simulink model "s_c_nbe_m1k"  (R2016b)
settings: Solver=VariableStepAuto  StartTime=0.0  StopTime=1000  RelTol=1e-3  EnableMultiTasking=on
undefined symbols (not defined in the file): Coeffs, fft_stages, n_taps, output_bits, pfb_coeff_gen_calc, xengbits
libraries: xbsIndex_r4 x23639, casper_library_misc x65, casper_library_scopes x4, xbsReplacements_r4 x4, xps_library x3
(part 142 of 198)

== system s_c_nbe_m1k/DDC/dec_fir_async2/fir_col_async8/fir_tap7 ==
  a : Inport
  b : Inport  Port=2
  c : Inport  Port=3
  d : Inport  Port=4
  dv_in : Inport  Port=5
  AddSub0 : xbsIndex_r4/AddSub  mode=Addition  use_carryin=off  use_carryout=off  en=off  latency=add_latency  precision=Full  arith_type="Signed  (2's comp)"  n_bits=18  bin_pt=16  quantization=Truncate  overflow=Wrap  use_behavioral_HDL=on  hw_selection=Fabric  pipelined=off  use_rpm=on  dbl_ovrd=off  block_type=addsub
  AddSub1 : xbsIndex_r4/AddSub  mode=Addition  use_carryin=off  use_carryout=off  en=off  latency=add_latency  precision=Full  arith_type="Signed  (2's comp)"  n_bits=18  bin_pt=16  quantization=Truncate  overflow=Wrap  use_behavioral_HDL=on  hw_selection=Fabric  pipelined=off  use_rpm=on  dbl_ovrd=off  block_type=addsub
  Mult0 : xbsIndex_r4/Mult  precision=Full  arith_type="Signed  (2's comp)"  n_bits=18  bin_pt=17  quantization=Truncate  overflow=Wrap  en=off  latency=mult_latency  use_behavioral_HDL=on  opt=Speed  use_embedded=on  optimum_pipeline=off  pipeline=on  dbl_ovrd=off  use_rpm=off  placement_style=Rectangular shape  block_type=mult
  Mult1 : xbsIndex_r4/Mult  precision=Full  arith_type="Signed  (2's comp)"  n_bits=18  bin_pt=17  quantization=Truncate  overflow=Wrap  en=off  latency=mult_latency  use_behavioral_HDL=on  opt=Speed  use_embedded=on  optimum_pipeline=off  pipeline=on  dbl_ovrd=off  use_rpm=off  placement_style=Rectangular shape  block_type=mult
  Register{0..3} (4 alike) : xbsIndex_r4/Register  init=0  rst=off  en=on  dbl_ovrd=off  block_type=register
  coefficient : xbsIndex_r4/Constant  const=factor  gui_display_data_type=Fixed-point  arith_type=Signed (2's comp)  n_bits=coeff_bit_width  bin_pt=coeff_bin_pt  preci_type=Single  exp_width=8  frac_width=24  explicit_period=on  period=1  equ=P=C  opselect=C  inp2=PCIN>>17  opr=+  inp1=P  carry=CIN  dbl_ovrd=off  block_type=constant
  a_out : Outport
  b_out : Outport  Port=2
  c_out : Outport  Port=3
  d_out : Outport  Port=4
  real : Outport  Port=5
  imag : Outport  Port=6
  wires:
  dv_in/1 -> Register0/2, Register1/2, Register2/2, Register3/2
  d/1 -> AddSub1/2, Register3/1
  c/1 -> AddSub0/2, Register2/1
  b/1 -> AddSub1/1, Register1/1
  a/1 -> AddSub0/1, Register0/1
  Register0/1 -> a_out/1
  Register1/1 -> b_out/1
  Register2/1 -> c_out/1
  coefficient/1 -> Mult0/1, Mult1/1
  Register3/1 -> d_out/1
  AddSub0/1 -> Mult0/2
  Mult0/1 -> real/1
  AddSub1/1 -> Mult1/2
  Mult1/1 -> imag/1

== system s_c_nbe_m1k/DDC/dec_fir_async2/fir_col_async8/fir_tap8 ==
  a : Inport
  b : Inport  Port=2
  c : Inport  Port=3
  d : Inport  Port=4
  dv_in : Inport  Port=5
  AddSub0 : xbsIndex_r4/AddSub  mode=Addition  use_carryin=off  use_carryout=off  en=off  latency=add_latency  precision=Full  arith_type="Signed  (2's comp)"  n_bits=18  bin_pt=16  quantization=Truncate  overflow=Wrap  use_behavioral_HDL=on  hw_selection=Fabric  pipelined=off  use_rpm=on  dbl_ovrd=off  block_type=addsub
  AddSub1 : xbsIndex_r4/AddSub  mode=Addition  use_carryin=off  use_carryout=off  en=off  latency=add_latency  precision=Full  arith_type="Signed  (2's comp)"  n_bits=18  bin_pt=16  quantization=Truncate  overflow=Wrap  use_behavioral_HDL=on  hw_selection=Fabric  pipelined=off  use_rpm=on  dbl_ovrd=off  block_type=addsub
  Mult0 : xbsIndex_r4/Mult  precision=Full  arith_type="Signed  (2's comp)"  n_bits=18  bin_pt=17  quantization=Truncate  overflow=Wrap  en=off  latency=mult_latency  use_behavioral_HDL=on  opt=Speed  use_embedded=on  optimum_pipeline=off  pipeline=on  dbl_ovrd=off  use_rpm=off  placement_style=Rectangular shape  block_type=mult
  Mult1 : xbsIndex_r4/Mult  precision=Full  arith_type="Signed  (2's comp)"  n_bits=18  bin_pt=17  quantization=Truncate  overflow=Wrap  en=off  latency=mult_latency  use_behavioral_HDL=on  opt=Speed  use_embedded=on  optimum_pipeline=off  pipeline=on  dbl_ovrd=off  use_rpm=off  placement_style=Rectangular shape  block_type=mult
  Register{0..3} (4 alike) : xbsIndex_r4/Register  init=0  rst=off  en=on  dbl_ovrd=off  block_type=register
  coefficient : xbsIndex_r4/Constant  const=factor  gui_display_data_type=Fixed-point  arith_type=Signed (2's comp)  n_bits=coeff_bit_width  bin_pt=coeff_bin_pt  preci_type=Single  exp_width=8  frac_width=24  explicit_period=on  period=1  equ=P=C  opselect=C  inp2=PCIN>>17  opr=+  inp1=P  carry=CIN  dbl_ovrd=off  block_type=constant
  a_out : Outport
  b_out : Outport  Port=2
  c_out : Outport  Port=3
  d_out : Outport  Port=4
  real : Outport  Port=5
  imag : Outport  Port=6
  wires:
  dv_in/1 -> Register0/2, Register1/2, Register2/2, Register3/2
  d/1 -> AddSub1/2, Register3/1
  c/1 -> AddSub0/2, Register2/1
  b/1 -> AddSub1/1, Register1/1
  a/1 -> AddSub0/1, Register0/1
  Register0/1 -> a_out/1
  Register1/1 -> b_out/1
  Register2/1 -> c_out/1
  coefficient/1 -> Mult0/1, Mult1/1
  Register3/1 -> d_out/1
  AddSub0/1 -> Mult0/2
  Mult0/1 -> real/1
  AddSub1/1 -> Mult1/2
  Mult1/1 -> imag/1

== system s_c_nbe_m1k/DDC/dec_fir_async2/fir_col_async8/fir_tap9 ==
  a : Inport
  b : Inport  Port=2
  c : Inport  Port=3
  d : Inport  Port=4
  dv_in : Inport  Port=5
  AddSub0 : xbsIndex_r4/AddSub  mode=Addition  use_carryin=off  use_carryout=off  en=off  latency=add_latency  precision=Full  arith_type="Signed  (2's comp)"  n_bits=18  bin_pt=16  quantization=Truncate  overflow=Wrap  use_behavioral_HDL=on  hw_selection=Fabric  pipelined=off  use_rpm=on  dbl_ovrd=off  block_type=addsub
  AddSub1 : xbsIndex_r4/AddSub  mode=Addition  use_carryin=off  use_carryout=off  en=off  latency=add_latency  precision=Full  arith_type="Signed  (2's comp)"  n_bits=18  bin_pt=16  quantization=Truncate  overflow=Wrap  use_behavioral_HDL=on  hw_selection=Fabric  pipelined=off  use_rpm=on  dbl_ovrd=off  block_type=addsub
  Mult0 : xbsIndex_r4/Mult  precision=Full  arith_type="Signed  (2's comp)"  n_bits=18  bin_pt=17  quantization=Truncate  overflow=Wrap  en=off  latency=mult_latency  use_behavioral_HDL=on  opt=Speed  use_embedded=on  optimum_pipeline=off  pipeline=on  dbl_ovrd=off  use_rpm=off  placement_style=Rectangular shape  block_type=mult
  Mult1 : xbsIndex_r4/Mult  precision=Full  arith_type="Signed  (2's comp)"  n_bits=18  bin_pt=17  quantization=Truncate  overflow=Wrap  en=off  latency=mult_latency  use_behavioral_HDL=on  opt=Speed  use_embedded=on  optimum_pipeline=off  pipeline=on  dbl_ovrd=off  use_rpm=off  placement_style=Rectangular shape  block_type=mult
  Register{0..3} (4 alike) : xbsIndex_r4/Register  init=0  rst=off  en=on  dbl_ovrd=off  block_type=register
  coefficient : xbsIndex_r4/Constant  const=factor  gui_display_data_type=Fixed-point  arith_type=Signed (2's comp)  n_bits=coeff_bit_width  bin_pt=coeff_bin_pt  preci_type=Single  exp_width=8  frac_width=24  explicit_period=on  period=1  equ=P=C  opselect=C  inp2=PCIN>>17  opr=+  inp1=P  carry=CIN  dbl_ovrd=off  block_type=constant
  a_out : Outport
  b_out : Outport  Port=2
  c_out : Outport  Port=3
  d_out : Outport  Port=4
  real : Outport  Port=5
  imag : Outport  Port=6
  wires:
  dv_in/1 -> Register0/2, Register1/2, Register2/2, Register3/2
  d/1 -> AddSub1/2, Register3/1
  c/1 -> AddSub0/2, Register2/1
  b/1 -> AddSub1/1, Register1/1
  a/1 -> AddSub0/1, Register0/1
  Register0/1 -> a_out/1
  Register1/1 -> b_out/1
  Register2/1 -> c_out/1
  coefficient/1 -> Mult0/1, Mult1/1
  Register3/1 -> d_out/1
  AddSub0/1 -> Mult0/2
  Mult0/1 -> real/1
  AddSub1/1 -> Mult1/2
  Mult1/1 -> imag/1

== system s_c_nbe_m1k/DDC/dec_fir_async3/convert_of/convert ==
  note: (ones_bit & 1) -> round-to-even
      | (ones_bit ^ 1) -> round-to-odd
      | (sign_bit & 1)-> round-to-zero
      | (sign_bit ^ 1) -> round-to-inf
      | (X ~| 1) -> round half down
      | (X | 1) -> round half up
  in : Inport
  Concat : xbsIndex_r4/Concat  num_inputs=2  dbl_ovrd=off  block_type=concat
      settings: block_version=10.1.3
  Constant : xbsIndex_r4/Constant  const=1  gui_display_data_type=Fixed-point  arith_type=Unsigned  n_bits=1  bin_pt=0  preci_type=Single  exp_width=8  frac_width=24  explicit_period=off  period=1  equ=P=C  opselect=C  inp2=PCIN>>17  opr=+  inp1=P  carry=CIN  dbl_ovrd=off  block_type=constant
  Reinterpret : xbsIndex_r4/Reinterpret  force_arith_type=on  arith_type=Unsigned  force_bin_pt=on  bin_pt=0  block_type=reinterpret
      settings: infoedit="Changes signal type without altering the binary representation.   You can changed the signal between signed and unsigned, and relocate the binary point.<P><P>Hardware notes: In hardware this block costs nothing.<P><P>Example:  Suppose the input is 6 bits wide, signed, with 2 fractional bits, and the output is forced to unsigned with 0 fractional bits.  Then an input of -2.0 (1110.00 in binary 2's complement) becomes an output of 56 (111000 in binary)."  block_version=10.1.3
  adder : xbsIndex_r4/AddSub  mode=Addition  use_carryin=off  use_carryout=off  en=off  latency=2  precision=User Defined  arith_type="Signed  (2's comp)"  n_bits=18  bin_pt=17  quantization=Truncate  overflow=Saturate  use_behavioral_HDL=off  hw_selection=Fabric  pipelined=on  use_rpm=on  dbl_ovrd=off  block_type=addsub
      settings: xl_area=[0, 0, 0, 0, 0, 0, 0]  block_version=10.1.3
  almost_half : xbsIndex_r4/Constant  const=131071  gui_display_data_type=Fixed-point  arith_type=Unsigned  n_bits=35  bin_pt=0  preci_type=Single  exp_width=8  frac_width=24  explicit_period=off  period=1  equ=P=C  opselect=C  inp2=PCIN>>17  opr=+  inp1=P  carry=CIN  dbl_ovrd=off  block_type=constant
  bit : xbsIndex_r4/Slice  nbits=1  boolean_output=off  mode=Lower Bit Location + Width  bit1=0  base1=MSB of Input  bit0=0  base0=MSB of Input  dbl_ovrd=off  block_type=slice
      settings: infoedit="Extracts a given range of bits from each input sample and presents it at the output.  The output type is ordinarily unsigned with binary point at zero, but can be Boolean when the slice is one bit wide.<P><P>Hardware notes: In hardware this block costs nothing."  block_version=10.1.3
  force1 : xbsIndex_r4/Reinterpret  force_arith_type=on  arith_type="Signed  (2's comp)"  force_bin_pt=on  bin_pt=35  block_type=reinterpret
      settings: infoedit="Changes signal type without altering the binary representation.   You can changed the signal between signed and unsigned, and relocate the binary point.<P><P>Hardware notes: In hardware this block costs nothing.<P><P>Example:  Suppose the input is 6 bits wide, signed, with 2 fractional bits, and the output is forced to unsigned with 0 fractional bits.  Then an input of -2.0 (1110.00 in binary 2's complement) becomes an output of 56 (111000 in binary)."  block_version=10.1.3
  force2 : xbsIndex_r4/Reinterpret  force_arith_type=off  arith_type="Signed  (2's comp)"  force_bin_pt=on  bin_pt=35  block_type=reinterpret
      settings: infoedit="Changes signal type without altering the binary representation.   You can changed the signal between signed and unsigned, and relocate the binary point.<P><P>Hardware notes: In hardware this block costs nothing.<P><P>Example:  Suppose the input is 6 bits wide, signed, with 2 fractional bits, and the output is forced to unsigned with 0 fractional bits.  Then an input of -2.0 (1110.00 in binary 2's complement) becomes an output of 56 (111000 in binary)."  block_version=10.1.3
  tweak_op : xbsIndex_r4/Logical  logical_function=XOR  inputs=2  en=off  latency=0  precision=Full  arith_type=Unsigned  n_bits=8  bin_pt=2  align_bp=on  dbl_ovrd=off  block_type=logical
      settings: xl_area=[0, 0, 0, 0, 0, 0, 0]
  out : Outport
  wires:
  adder/1 -> out/1
  force2/1 -> adder/2
  force1/1 -> adder/1
  Reinterpret/1 -> Concat/1
  Concat/1 -> force1/1
  in/1 -> bit/1, Reinterpret/1
  almost_half/1 -> force2/1
  bit/1 -> tweak_op/1
  Constant/1 -> tweak_op/2
  tweak_op/1 -> Concat/2

== system s_c_nbe_m1k/DDC/dec_fir_async3/convert_of1/convert ==
  note: (ones_bit & 1) -> round-to-even
      | (ones_bit ^ 1) -> round-to-odd
      | (sign_bit & 1)-> round-to-zero
      | (sign_bit ^ 1) -> round-to-inf
      | (X ~| 1) -> round half down
      | (X | 1) -> round half up
  in : Inport
  Concat : xbsIndex_r4/Concat  num_inputs=2  dbl_ovrd=off  block_type=concat
      settings: block_version=10.1.3
  Constant : xbsIndex_r4/Constant  const=1  gui_display_data_type=Fixed-point  arith_type=Unsigned  n_bits=1  bin_pt=0  preci_type=Single  exp_width=8  frac_width=24  explicit_period=off  period=1  equ=P=C  opselect=C  inp2=PCIN>>17  opr=+  inp1=P  carry=CIN  dbl_ovrd=off  block_type=constant
  Reinterpret : xbsIndex_r4/Reinterpret  force_arith_type=on  arith_type=Unsigned  force_bin_pt=on  bin_pt=0  block_type=reinterpret
      settings: infoedit="Changes signal type without altering the binary representation.   You can changed the signal between signed and unsigned, and relocate the binary point.<P><P>Hardware notes: In hardware this block costs nothing.<P><P>Example:  Suppose the input is 6 bits wide, signed, with 2 fractional bits, and the output is forced to unsigned with 0 fractional bits.  Then an input of -2.0 (1110.00 in binary 2's complement) becomes an output of 56 (111000 in binary)."  block_version=10.1.3
  adder : xbsIndex_r4/AddSub  mode=Addition  use_carryin=off  use_carryout=off  en=off  latency=2  precision=User Defined  arith_type="Signed  (2's comp)"  n_bits=18  bin_pt=17  quantization=Truncate  overflow=Saturate  use_behavioral_HDL=off  hw_selection=Fabric  pipelined=on  use_rpm=on  dbl_ovrd=off  block_type=addsub
      settings: xl_area=[0, 0, 0, 0, 0, 0, 0]  block_version=10.1.3
  almost_half : xbsIndex_r4/Constant  const=131071  gui_display_data_type=Fixed-point  arith_type=Unsigned  n_bits=35  bin_pt=0  preci_type=Single  exp_width=8  frac_width=24  explicit_period=off  period=1  equ=P=C  opselect=C  inp2=PCIN>>17  opr=+  inp1=P  carry=CIN  dbl_ovrd=off  block_type=constant
  bit : xbsIndex_r4/Slice  nbits=1  boolean_output=off  mode=Lower Bit Location + Width  bit1=0  base1=MSB of Input  bit0=0  base0=MSB of Input  dbl_ovrd=off  block_type=slice
      settings: infoedit="Extracts a given range of bits from each input sample and presents it at the output.  The output type is ordinarily unsigned with binary point at zero, but can be Boolean when the slice is one bit wide.<P><P>Hardware notes: In hardware this block costs nothing."  block_version=10.1.3
  force1 : xbsIndex_r4/Reinterpret  force_arith_type=on  arith_type="Signed  (2's comp)"  force_bin_pt=on  bin_pt=35  block_type=reinterpret
      settings: infoedit="Changes signal type without altering the binary representation.   You can changed the signal between signed and unsigned, and relocate the binary point.<P><P>Hardware notes: In hardware this block costs nothing.<P><P>Example:  Suppose the input is 6 bits wide, signed, with 2 fractional bits, and the output is forced to unsigned with 0 fractional bits.  Then an input of -2.0 (1110.00 in binary 2's complement) becomes an output of 56 (111000 in binary)."  block_version=10.1.3
  force2 : xbsIndex_r4/Reinterpret  force_arith_type=off  arith_type="Signed  (2's comp)"  force_bin_pt=on  bin_pt=35  block_type=reinterpret
      settings: infoedit="Changes signal type without altering the binary representation.   You can changed the signal between signed and unsigned, and relocate the binary point.<P><P>Hardware notes: In hardware this block costs nothing.<P><P>Example:  Suppose the input is 6 bits wide, signed, with 2 fractional bits, and the output is forced to unsigned with 0 fractional bits.  Then an input of -2.0 (1110.00 in binary 2's complement) becomes an output of 56 (111000 in binary)."  block_version=10.1.3
  tweak_op : xbsIndex_r4/Logical  logical_function=XOR  inputs=2  en=off  latency=0  precision=Full  arith_type=Unsigned  n_bits=8  bin_pt=2  align_bp=on  dbl_ovrd=off  block_type=logical
      settings: xl_area=[0, 0, 0, 0, 0, 0, 0]
  out : Outport
  wires:
  tweak_op/1 -> Concat/2
  Constant/1 -> tweak_op/2
  bit/1 -> tweak_op/1
  almost_half/1 -> force2/1
  in/1 -> Reinterpret/1, bit/1
  Concat/1 -> force1/1
  Reinterpret/1 -> Concat/1
  force1/1 -> adder/1
  force2/1 -> adder/2
  adder/1 -> out/1

== system s_c_nbe_m1k/DDC/dec_fir_async3/fir_col_async1/adder_tree1 ==
  sync : Inport
  din1 : Inport  Port=2
  din2 : Inport  Port=3
  din3 : Inport  Port=4
  din4 : Inport  Port=5
  din5 : Inport  Port=6
  din6 : Inport  Port=7
  din7 : Inport  Port=8
  din8 : Inport  Port=9
  din9 : Inport  Port=10
  din10 : Inport  Port=11
  din11 : Inport  Port=12
  din12 : Inport  Port=13
  din13 : Inport  Port=14
  din14 : Inport  Port=15
  din15 : Inport  Port=16
  din16 : Inport  Port=17
  addr{1..8} (8 alike) : xbsIndex_r4/AddSub  mode=Addition  use_carryin=off  use_carryout=off  en=off  latency=7  precision=Full  arith_type=Unsigned  n_bits=16  bin_pt=14  quantization=Truncate  overflow=Wrap  use_behavioral_HDL=on  hw_selection=DSP48  pipelined=on  use_rpm=on  dbl_ovrd=off  block_type=addsub
  addr{9..15} (7 alike) : xbsIndex_r4/AddSub  mode=Addition  use_carryin=off  use_carryout=off  en=off  latency=7  precision=Full  arith_type=Unsigned  n_bits=16  bin_pt=14  quantization=Truncate  overflow=Wrap  use_behavioral_HDL=off  hw_selection=DSP48  pipelined=on  use_rpm=on  dbl_ovrd=off  block_type=addsub
  sync_delay : xbsIndex_r4/Delay  rst=off  infoeditControl=Selection of Reset will increase slice count due to use of real FFs and instead of SRLs  en=off  latency=28  reg_retiming=on  dbl_ovrd=off  block_type=delay
      settings: block_version=11.4
  sync_out : Outport
  dout : Outport  Port=2
  wires:
  addr15/1 -> dout/1
  addr14/1 -> addr15/2
  addr13/1 -> addr15/1
  addr12/1 -> addr14/2
  addr11/1 -> addr14/1
  addr10/1 -> addr13/2
  addr9/1 -> addr13/1
  addr8/1 -> addr12/2
  addr7/1 -> addr12/1
  addr6/1 -> addr11/2
  addr5/1 -> addr11/1
  addr4/1 -> addr10/2
  addr3/1 -> addr10/1
  addr2/1 -> addr9/2
  addr1/1 -> addr9/1
  din16/1 -> addr8/2
  din15/1 -> addr8/1
  din14/1 -> addr7/2
  din13/1 -> addr7/1
  din12/1 -> addr6/2
  din11/1 -> addr6/1
  din10/1 -> addr5/2
  din9/1 -> addr5/1
  din8/1 -> addr4/2
  din7/1 -> addr4/1
  din6/1 -> addr3/2
  din5/1 -> addr3/1
  din4/1 -> addr2/2
  din3/1 -> addr2/1
  din2/1 -> addr1/2
  din1/1 -> addr1/1
  sync_delay/1 -> sync_out/1
  sync/1 -> sync_delay/1

== system s_c_nbe_m1k/DDC/dec_fir_async3/fir_col_async1/adder_tree2 ==
  sync : Inport
  din1 : Inport  Port=2
  din2 : Inport  Port=3
  din3 : Inport  Port=4
  din4 : Inport  Port=5
  din5 : Inport  Port=6
  din6 : Inport  Port=7
  din7 : Inport  Port=8
  din8 : Inport  Port=9
  din9 : Inport  Port=10
  din10 : Inport  Port=11
  din11 : Inport  Port=12
  din12 : Inport  Port=13
  din13 : Inport  Port=14
  din14 : Inport  Port=15
  din15 : Inport  Port=16
  din16 : Inport  Port=17
  addr{1..8} (8 alike) : xbsIndex_r4/AddSub  mode=Addition  use_carryin=off  use_carryout=off  en=off  latency=7  precision=Full  arith_type=Unsigned  n_bits=16  bin_pt=14  quantization=Truncate  overflow=Wrap  use_behavioral_HDL=on  hw_selection=DSP48  pipelined=on  use_rpm=on  dbl_ovrd=off  block_type=addsub
  addr{9..15} (7 alike) : xbsIndex_r4/AddSub  mode=Addition  use_carryin=off  use_carryout=off  en=off  latency=7  precision=Full  arith_type=Unsigned  n_bits=16  bin_pt=14  quantization=Truncate  overflow=Wrap  use_behavioral_HDL=off  hw_selection=DSP48  pipelined=on  use_rpm=on  dbl_ovrd=off  block_type=addsub
  sync_delay : xbsIndex_r4/Delay  rst=off  infoeditControl=Selection of Reset will increase slice count due to use of real FFs and instead of SRLs  en=off  latency=28  reg_retiming=on  dbl_ovrd=off  block_type=delay
      settings: block_version=11.4
  sync_out : Outport
  dout : Outport  Port=2
  wires:
  addr15/1 -> dout/1
  addr14/1 -> addr15/2
  addr13/1 -> addr15/1
  addr12/1 -> addr14/2
  addr11/1 -> addr14/1
  addr10/1 -> addr13/2
  addr9/1 -> addr13/1
  addr8/1 -> addr12/2
  addr7/1 -> addr12/1
  addr6/1 -> addr11/2
  addr5/1 -> addr11/1
  addr4/1 -> addr10/2
  addr3/1 -> addr10/1
  addr2/1 -> addr9/2
  addr1/1 -> addr9/1
  din16/1 -> addr8/2
  din15/1 -> addr8/1
  din14/1 -> addr7/2
  din13/1 -> addr7/1
  din12/1 -> addr6/2
  din11/1 -> addr6/1
  din10/1 -> addr5/2
  din9/1 -> addr5/1
  din8/1 -> addr4/2
  din7/1 -> addr4/1
  din6/1 -> addr3/2
  din5/1 -> addr3/1
  din4/1 -> addr2/2
  din3/1 -> addr2/1
  din2/1 -> addr1/2
  din1/1 -> addr1/1
  sync_delay/1 -> sync_out/1
  sync/1 -> sync_delay/1

== system s_c_nbe_m1k/DDC/dec_fir_async3/fir_col_async1/fir_tap1 ==
  a : Inport
  b : Inport  Port=2
  c : Inport  Port=3
  d : Inport  Port=4
  dv_in : Inport  Port=5
  AddSub0 : xbsIndex_r4/AddSub  mode=Addition  use_carryin=off  use_carryout=off  en=off  latency=add_latency  precision=Full  arith_type="Signed  (2's comp)"  n_bits=18  bin_pt=16  quantization=Truncate  overflow=Wrap  use_behavioral_HDL=on  hw_selection=Fabric  pipelined=off  use_rpm=on  dbl_ovrd=off  block_type=addsub
  AddSub1 : xbsIndex_r4/AddSub  mode=Addition  use_carryin=off  use_carryout=off  en=off  latency=add_latency  precision=Full  arith_type="Signed  (2's comp)"  n_bits=18  bin_pt=16  quantization=Truncate  overflow=Wrap  use_behavioral_HDL=on  hw_selection=Fabric  pipelined=off  use_rpm=on  dbl_ovrd=off  block_type=addsub
  Mult0 : xbsIndex_r4/Mult  precision=Full  arith_type="Signed  (2's comp)"  n_bits=18  bin_pt=17  quantization=Truncate  overflow=Wrap  en=off  latency=mult_latency  use_behavioral_HDL=on  opt=Speed  use_embedded=on  optimum_pipeline=off  pipeline=on  dbl_ovrd=off  use_rpm=off  placement_style=Rectangular shape  block_type=mult
  Mult1 : xbsIndex_r4/Mult  precision=Full  arith_type="Signed  (2's comp)"  n_bits=18  bin_pt=17  quantization=Truncate  overflow=Wrap  en=off  latency=mult_latency  use_behavioral_HDL=on  opt=Speed  use_embedded=on  optimum_pipeline=off  pipeline=on  dbl_ovrd=off  use_rpm=off  placement_style=Rectangular shape  block_type=mult
  Register{0..3} (4 alike) : xbsIndex_r4/Register  init=0  rst=off  en=on  dbl_ovrd=off  block_type=register
  coefficient : xbsIndex_r4/Constant  const=factor  gui_display_data_type=Fixed-point  arith_type=Signed (2's comp)  n_bits=coeff_bit_width  bin_pt=coeff_bin_pt  preci_type=Single  exp_width=8  frac_width=24  explicit_period=on  period=1  equ=P=C  opselect=C  inp2=PCIN>>17  opr=+  inp1=P  carry=CIN  dbl_ovrd=off  block_type=constant
  a_out : Outport
  b_out : Outport  Port=2
  c_out : Outport  Port=3
  d_out : Outport  Port=4
  real : Outport  Port=5
  imag : Outport  Port=6
  wires:
  Mult1/1 -> imag/1
  AddSub1/1 -> Mult1/2
  Mult0/1 -> real/1
  AddSub0/1 -> Mult0/2
  Register3/1 -> d_out/1
  coefficient/1 -> Mult1/1, Mult0/1
  Register2/1 -> c_out/1
  Register1/1 -> b_out/1
  Register0/1 -> a_out/1
  a/1 -> Register0/1, AddSub0/1
  b/1 -> Register1/1, AddSub1/1
  c/1 -> Register2/1, AddSub0/2
  d/1 -> Register3/1, AddSub1/2
  dv_in/1 -> Register0/2, Register1/2, Register3/2, Register2/2

== system s_c_nbe_m1k/DDC/dec_fir_async3/fir_col_async1/fir_tap10 ==
  a : Inport
  b : Inport  Port=2
  c : Inport  Port=3
  d : Inport  Port=4
  dv_in : Inport  Port=5
  AddSub0 : xbsIndex_r4/AddSub  mode=Addition  use_carryin=off  use_carryout=off  en=off  latency=add_latency  precision=Full  arith_type="Signed  (2's comp)"  n_bits=18  bin_pt=16  quantization=Truncate  overflow=Wrap  use_behavioral_HDL=on  hw_selection=Fabric  pipelined=off  use_rpm=on  dbl_ovrd=off  block_type=addsub
  AddSub1 : xbsIndex_r4/AddSub  mode=Addition  use_carryin=off  use_carryout=off  en=off  latency=add_latency  precision=Full  arith_type="Signed  (2's comp)"  n_bits=18  bin_pt=16  quantization=Truncate  overflow=Wrap  use_behavioral_HDL=on  hw_selection=Fabric  pipelined=off  use_rpm=on  dbl_ovrd=off  block_type=addsub
  Mult0 : xbsIndex_r4/Mult  precision=Full  arith_type="Signed  (2's comp)"  n_bits=18  bin_pt=17  quantization=Truncate  overflow=Wrap  en=off  latency=mult_latency  use_behavioral_HDL=on  opt=Speed  use_embedded=on  optimum_pipeline=off  pipeline=on  dbl_ovrd=off  use_rpm=off  placement_style=Rectangular shape  block_type=mult
  Mult1 : xbsIndex_r4/Mult  precision=Full  arith_type="Signed  (2's comp)"  n_bits=18  bin_pt=17  quantization=Truncate  overflow=Wrap  en=off  latency=mult_latency  use_behavioral_HDL=on  opt=Speed  use_embedded=on  optimum_pipeline=off  pipeline=on  dbl_ovrd=off  use_rpm=off  placement_style=Rectangular shape  block_type=mult
  Register{0..3} (4 alike) : xbsIndex_r4/Register  init=0  rst=off  en=on  dbl_ovrd=off  block_type=register
  coefficient : xbsIndex_r4/Constant  const=factor  gui_display_data_type=Fixed-point  arith_type=Signed (2's comp)  n_bits=coeff_bit_width  bin_pt=coeff_bin_pt  preci_type=Single  exp_width=8  frac_width=24  explicit_period=on  period=1  equ=P=C  opselect=C  inp2=PCIN>>17  opr=+  inp1=P  carry=CIN  dbl_ovrd=off  block_type=constant
  a_out : Outport
  b_out : Outport  Port=2
  c_out : Outport  Port=3
  d_out : Outport  Port=4
  real : Outport  Port=5
  imag : Outport  Port=6
  wires:
  Mult1/1 -> imag/1
  AddSub1/1 -> Mult1/2
  Mult0/1 -> real/1
  AddSub0/1 -> Mult0/2
  Register3/1 -> d_out/1
  coefficient/1 -> Mult1/1, Mult0/1
  Register2/1 -> c_out/1
  Register1/1 -> b_out/1
  Register0/1 -> a_out/1
  a/1 -> Register0/1, AddSub0/1
  b/1 -> Register1/1, AddSub1/1
  c/1 -> Register2/1, AddSub0/2
  d/1 -> Register3/1, AddSub1/2
  dv_in/1 -> Register3/2, Register2/2, Register1/2, Register0/2

== system s_c_nbe_m1k/DDC/dec_fir_async3/fir_col_async1/fir_tap11 ==
  a : Inport
  b : Inport  Port=2
  c : Inport  Port=3
  d : Inport  Port=4
  dv_in : Inport  Port=5
  AddSub0 : xbsIndex_r4/AddSub  mode=Addition  use_carryin=off  use_carryout=off  en=off  latency=add_latency  precision=Full  arith_type="Signed  (2's comp)"  n_bits=18  bin_pt=16  quantization=Truncate  overflow=Wrap  use_behavioral_HDL=on  hw_selection=Fabric  pipelined=off  use_rpm=on  dbl_ovrd=off  block_type=addsub
  AddSub1 : xbsIndex_r4/AddSub  mode=Addition  use_carryin=off  use_carryout=off  en=off  latency=add_latency  precision=Full  arith_type="Signed  (2's comp)"  n_bits=18  bin_pt=16  quantization=Truncate  overflow=Wrap  use_behavioral_HDL=on  hw_selection=Fabric  pipelined=off  use_rpm=on  dbl_ovrd=off  block_type=addsub
  Mult0 : xbsIndex_r4/Mult  precision=Full  arith_type="Signed  (2's comp)"  n_bits=18  bin_pt=17  quantization=Truncate  overflow=Wrap  en=off  latency=mult_latency  use_behavioral_HDL=on  opt=Speed  use_embedded=on  optimum_pipeline=off  pipeline=on  dbl_ovrd=off  use_rpm=off  placement_style=Rectangular shape  block_type=mult
  Mult1 : xbsIndex_r4/Mult  precision=Full  arith_type="Signed  (2's comp)"  n_bits=18  bin_pt=17  quantization=Truncate  overflow=Wrap  en=off  latency=mult_latency  use_behavioral_HDL=on  opt=Speed  use_embedded=on  optimum_pipeline=off  pipeline=on  dbl_ovrd=off  use_rpm=off  placement_style=Rectangular shape  block_type=mult
  Register{0..3} (4 alike) : xbsIndex_r4/Register  init=0  rst=off  en=on  dbl_ovrd=off  block_type=register
  coefficient : xbsIndex_r4/Constant  const=factor  gui_display_data_type=Fixed-point  arith_type=Signed (2's comp)  n_bits=coeff_bit_width  bin_pt=coeff_bin_pt  preci_type=Single  exp_width=8  frac_width=24  explicit_period=on  period=1  equ=P=C  opselect=C  inp2=PCIN>>17  opr=+  inp1=P  carry=CIN  dbl_ovrd=off  block_type=constant
  a_out : Outport
  b_out : Outport  Port=2
  c_out : Outport  Port=3
  d_out : Outport  Port=4
  real : Outport  Port=5
  imag : Outport  Port=6
  wires:
  Mult1/1 -> imag/1
  AddSub1/1 -> Mult1/2
  Mult0/1 -> real/1
  AddSub0/1 -> Mult0/2
  Register3/1 -> d_out/1
  coefficient/1 -> Mult1/1, Mult0/1
  Register2/1 -> c_out/1
  Register1/1 -> b_out/1
  Register0/1 -> a_out/1
  a/1 -> Register0/1, AddSub0/1
  b/1 -> Register1/1, AddSub1/1
  c/1 -> Register2/1, AddSub0/2
  d/1 -> Register3/1, AddSub1/2
  dv_in/1 -> Register3/2, Register2/2, Register1/2, Register0/2

== system s_c_nbe_m1k/DDC/dec_fir_async3/fir_col_async1/fir_tap12 ==
  a : Inport
  b : Inport  Port=2
  c : Inport  Port=3
  d : Inport  Port=4
  dv_in : Inport  Port=5
  AddSub0 : xbsIndex_r4/AddSub  mode=Addition  use_carryin=off  use_carryout=off  en=off  latency=add_latency  precision=Full  arith_type="Signed  (2's comp)"  n_bits=18  bin_pt=16  quantization=Truncate  overflow=Wrap  use_behavioral_HDL=on  hw_selection=Fabric  pipelined=off  use_rpm=on  dbl_ovrd=off  block_type=addsub
  AddSub1 : xbsIndex_r4/AddSub  mode=Addition  use_carryin=off  use_carryout=off  en=off  latency=add_latency  precision=Full  arith_type="Signed  (2's comp)"  n_bits=18  bin_pt=16  quantization=Truncate  overflow=Wrap  use_behavioral_HDL=on  hw_selection=Fabric  pipelined=off  use_rpm=on  dbl_ovrd=off  block_type=addsub
  Mult0 : xbsIndex_r4/Mult  precision=Full  arith_type="Signed  (2's comp)"  n_bits=18  bin_pt=17  quantization=Truncate  overflow=Wrap  en=off  latency=mult_latency  use_behavioral_HDL=on  opt=Speed  use_embedded=on  optimum_pipeline=off  pipeline=on  dbl_ovrd=off  use_rpm=off  placement_style=Rectangular shape  block_type=mult
  Mult1 : xbsIndex_r4/Mult  precision=Full  arith_type="Signed  (2's comp)"  n_bits=18  bin_pt=17  quantization=Truncate  overflow=Wrap  en=off  latency=mult_latency  use_behavioral_HDL=on  opt=Speed  use_embedded=on  optimum_pipeline=off  pipeline=on  dbl_ovrd=off  use_rpm=off  placement_style=Rectangular shape  block_type=mult
  Register{0..3} (4 alike) : xbsIndex_r4/Register  init=0  rst=off  en=on  dbl_ovrd=off  block_type=register
  coefficient : xbsIndex_r4/Constant  const=factor  gui_display_data_type=Fixed-point  arith_type=Signed (2's comp)  n_bits=coeff_bit_width  bin_pt=coeff_bin_pt  preci_type=Single  exp_width=8  frac_width=24  explicit_period=on  period=1  equ=P=C  opselect=C  inp2=PCIN>>17  opr=+  inp1=P  carry=CIN  dbl_ovrd=off  block_type=constant
  a_out : Outport
  b_out : Outport  Port=2
  c_out : Outport  Port=3
  d_out : Outport  Port=4
  real : Outport  Port=5
  imag : Outport  Port=6
  wires:
  Mult1/1 -> imag/1
  AddSub1/1 -> Mult1/2
  Mult0/1 -> real/1
  AddSub0/1 -> Mult0/2
  Register3/1 -> d_out/1
  coefficient/1 -> Mult1/1, Mult0/1
  Register2/1 -> c_out/1
  Register1/1 -> b_out/1
  Register0/1 -> a_out/1
  a/1 -> Register0/1, AddSub0/1
  b/1 -> Register1/1, AddSub1/1
  c/1 -> Register2/1, AddSub0/2
  d/1 -> Register3/1, AddSub1/2
  dv_in/1 -> Register3/2, Register2/2, Register1/2, Register0/2

== system s_c_nbe_m1k/DDC/dec_fir_async3/fir_col_async1/fir_tap13 ==
  a : Inport
  b : Inport  Port=2
  c : Inport  Port=3
  d : Inport  Port=4
  dv_in : Inport  Port=5
  AddSub0 : xbsIndex_r4/AddSub  mode=Addition  use_carryin=off  use_carryout=off  en=off  latency=add_latency  precision=Full  arith_type="Signed  (2's comp)"  n_bits=18  bin_pt=16  quantization=Truncate  overflow=Wrap  use_behavioral_HDL=on  hw_selection=Fabric  pipelined=off  use_rpm=on  dbl_ovrd=off  block_type=addsub
  AddSub1 : xbsIndex_r4/AddSub  mode=Addition  use_carryin=off  use_carryout=off  en=off  latency=add_latency  precision=Full  arith_type="Signed  (2's comp)"  n_bits=18  bin_pt=16  quantization=Truncate  overflow=Wrap  use_behavioral_HDL=on  hw_selection=Fabric  pipelined=off  use_rpm=on  dbl_ovrd=off  block_type=addsub
  Mult0 : xbsIndex_r4/Mult  precision=Full  arith_type="Signed  (2's comp)"  n_bits=18  bin_pt=17  quantization=Truncate  overflow=Wrap  en=off  latency=mult_latency  use_behavioral_HDL=on  opt=Speed  use_embedded=on  optimum_pipeline=off  pipeline=on  dbl_ovrd=off  use_rpm=off  placement_style=Rectangular shape  block_type=mult
  Mult1 : xbsIndex_r4/Mult  precision=Full  arith_type="Signed  (2's comp)"  n_bits=18  bin_pt=17  quantization=Truncate  overflow=Wrap  en=off  latency=mult_latency  use_behavioral_HDL=on  opt=Speed  use_embedded=on  optimum_pipeline=off  pipeline=on  dbl_ovrd=off  use_rpm=off  placement_style=Rectangular shape  block_type=mult
  Register{0..3} (4 alike) : xbsIndex_r4/Register  init=0  rst=off  en=on  dbl_ovrd=off  block_type=register
  coefficient : xbsIndex_r4/Constant  const=factor  gui_display_data_type=Fixed-point  arith_type=Signed (2's comp)  n_bits=coeff_bit_width  bin_pt=coeff_bin_pt  preci_type=Single  exp_width=8  frac_width=24  explicit_period=on  period=1  equ=P=C  opselect=C  inp2=PCIN>>17  opr=+  inp1=P  carry=CIN  dbl_ovrd=off  block_type=constant
  a_out : Outport
  b_out : Outport  Port=2
  c_out : Outport  Port=3
  d_out : Outport  Port=4
  real : Outport  Port=5
  imag : Outport  Port=6
  wires:
  Mult1/1 -> imag/1
  AddSub1/1 -> Mult1/2
  Mult0/1 -> real/1
  AddSub0/1 -> Mult0/2
  Register3/1 -> d_out/1
  coefficient/1 -> Mult1/1, Mult0/1
  Register2/1 -> c_out/1
  Register1/1 -> b_out/1
  Register0/1 -> a_out/1
  a/1 -> Register0/1, AddSub0/1
  b/1 -> Register1/1, AddSub1/1
  c/1 -> Register2/1, AddSub0/2
  d/1 -> Register3/1, AddSub1/2
  dv_in/1 -> Register3/2, Register2/2, Register1/2, Register0/2

== system s_c_nbe_m1k/DDC/dec_fir_async3/fir_col_async1/fir_tap14 ==
  a : Inport
  b : Inport  Port=2
  c : Inport  Port=3
  d : Inport  Port=4
  dv_in : Inport  Port=5
  AddSub0 : xbsIndex_r4/AddSub  mode=Addition  use_carryin=off  use_carryout=off  en=off  latency=add_latency  precision=Full  arith_type="Signed  (2's comp)"  n_bits=18  bin_pt=16  quantization=Truncate  overflow=Wrap  use_behavioral_HDL=on  hw_selection=Fabric  pipelined=off  use_rpm=on  dbl_ovrd=off  block_type=addsub
  AddSub1 : xbsIndex_r4/AddSub  mode=Addition  use_carryin=off  use_carryout=off  en=off  latency=add_latency  precision=Full  arith_type="Signed  (2's comp)"  n_bits=18  bin_pt=16  quantization=Truncate  overflow=Wrap  use_behavioral_HDL=on  hw_selection=Fabric  pipelined=off  use_rpm=on  dbl_ovrd=off  block_type=addsub
  Mult0 : xbsIndex_r4/Mult  precision=Full  arith_type="Signed  (2's comp)"  n_bits=18  bin_pt=17  quantization=Truncate  overflow=Wrap  en=off  latency=mult_latency  use_behavioral_HDL=on  opt=Speed  use_embedded=on  optimum_pipeline=off  pipeline=on  dbl_ovrd=off  use_rpm=off  placement_style=Rectangular shape  block_type=mult
  Mult1 : xbsIndex_r4/Mult  precision=Full  arith_type="Signed  (2's comp)"  n_bits=18  bin_pt=17  quantization=Truncate  overflow=Wrap  en=off  latency=mult_latency  use_behavioral_HDL=on  opt=Speed  use_embedded=on  optimum_pipeline=off  pipeline=on  dbl_ovrd=off  use_rpm=off  placement_style=Rectangular shape  block_type=mult
  Register{0..3} (4 alike) : xbsIndex_r4/Register  init=0  rst=off  en=on  dbl_ovrd=off  block_type=register
  coefficient : xbsIndex_r4/Constant  const=factor  gui_display_data_type=Fixed-point  arith_type=Signed (2's comp)  n_bits=coeff_bit_width  bin_pt=coeff_bin_pt  preci_type=Single  exp_width=8  frac_width=24  explicit_period=on  period=1  equ=P=C  opselect=C  inp2=PCIN>>17  opr=+  inp1=P  carry=CIN  dbl_ovrd=off  block_type=constant
  a_out : Outport
  b_out : Outport  Port=2
  c_out : Outport  Port=3
  d_out : Outport  Port=4
  real : Outport  Port=5
  imag : Outport  Port=6
  wires:
  Mult1/1 -> imag/1
  AddSub1/1 -> Mult1/2
  Mult0/1 -> real/1
  AddSub0/1 -> Mult0/2
  Register3/1 -> d_out/1
  coefficient/1 -> Mult1/1, Mult0/1
  Register2/1 -> c_out/1
  Register1/1 -> b_out/1
  Register0/1 -> a_out/1
  a/1 -> Register0/1, AddSub0/1
  b/1 -> Register1/1, AddSub1/1
  c/1 -> Register2/1, AddSub0/2
  d/1 -> Register3/1, AddSub1/2
  dv_in/1 -> Register3/2, Register2/2, Register1/2, Register0/2

== system s_c_nbe_m1k/DDC/dec_fir_async3/fir_col_async1/fir_tap15 ==
  a : Inport
  b : Inport  Port=2
  c : Inport  Port=3
  d : Inport  Port=4
  dv_in : Inport  Port=5
  AddSub0 : xbsIndex_r4/AddSub  mode=Addition  use_carryin=off  use_carryout=off  en=off  latency=add_latency  precision=Full  arith_type="Signed  (2's comp)"  n_bits=18  bin_pt=16  quantization=Truncate  overflow=Wrap  use_behavioral_HDL=on  hw_selection=Fabric  pipelined=off  use_rpm=on  dbl_ovrd=off  block_type=addsub
  AddSub1 : xbsIndex_r4/AddSub  mode=Addition  use_carryin=off  use_carryout=off  en=off  latency=add_latency  precision=Full  arith_type="Signed  (2's comp)"  n_bits=18  bin_pt=16  quantization=Truncate  overflow=Wrap  use_behavioral_HDL=on  hw_selection=Fabric  pipelined=off  use_rpm=on  dbl_ovrd=off  block_type=addsub
  Mult0 : xbsIndex_r4/Mult  precision=Full  arith_type="Signed  (2's comp)"  n_bits=18  bin_pt=17  quantization=Truncate  overflow=Wrap  en=off  latency=mult_latency  use_behavioral_HDL=on  opt=Speed  use_embedded=on  optimum_pipeline=off  pipeline=on  dbl_ovrd=off  use_rpm=off  placement_style=Rectangular shape  block_type=mult
  Mult1 : xbsIndex_r4/Mult  precision=Full  arith_type="Signed  (2's comp)"  n_bits=18  bin_pt=17  quantization=Truncate  overflow=Wrap  en=off  latency=mult_latency  use_behavioral_HDL=on  opt=Speed  use_embedded=on  optimum_pipeline=off  pipeline=on  dbl_ovrd=off  use_rpm=off  placement_style=Rectangular shape  block_type=mult
  Register{0..3} (4 alike) : xbsIndex_r4/Register  init=0  rst=off  en=on  dbl_ovrd=off  block_type=register
  coefficient : xbsIndex_r4/Constant  const=factor  gui_display_data_type=Fixed-point  arith_type=Signed (2's comp)  n_bits=coeff_bit_width  bin_pt=coeff_bin_pt  preci_type=Single  exp_width=8  frac_width=24  explicit_period=on  period=1  equ=P=C  opselect=C  inp2=PCIN>>17  opr=+  inp1=P  carry=CIN  dbl_ovrd=off  block_type=constant
  a_out : Outport
  b_out : Outport  Port=2
  c_out : Outport  Port=3
  d_out : Outport  Port=4
  real : Outport  Port=5
  imag : Outport  Port=6
  wires:
  Mult1/1 -> imag/1
  AddSub1/1 -> Mult1/2
  Mult0/1 -> real/1
  AddSub0/1 -> Mult0/2
  Register3/1 -> d_out/1
  coefficient/1 -> Mult1/1, Mult0/1
  Register2/1 -> c_out/1
  Register1/1 -> b_out/1
  Register0/1 -> a_out/1
  a/1 -> Register0/1, AddSub0/1
  b/1 -> Register1/1, AddSub1/1
  c/1 -> Register2/1, AddSub0/2
  d/1 -> Register3/1, AddSub1/2
  dv_in/1 -> Register3/2, Register2/2, Register1/2, Register0/2

== system s_c_nbe_m1k/DDC/dec_fir_async3/fir_col_async1/fir_tap16 ==
  a : Inport
  b : Inport  Port=2
  c : Inport  Port=3
  d : Inport  Port=4
  dv_in : Inport  Port=5
  AddSub0 : xbsIndex_r4/AddSub  mode=Addition  use_carryin=off  use_carryout=off  en=off  latency=add_latency  precision=Full  arith_type="Signed  (2's comp)"  n_bits=18  bin_pt=16  quantization=Truncate  overflow=Wrap  use_behavioral_HDL=on  hw_selection=Fabric  pipelined=off  use_rpm=on  dbl_ovrd=off  block_type=addsub
  AddSub1 : xbsIndex_r4/AddSub  mode=Addition  use_carryin=off  use_carryout=off  en=off  latency=add_latency  precision=Full  arith_type="Signed  (2's comp)"  n_bits=18  bin_pt=16  quantization=Truncate  overflow=Wrap  use_behavioral_HDL=on  hw_selection=Fabric  pipelined=off  use_rpm=on  dbl_ovrd=off  block_type=addsub
  Mult0 : xbsIndex_r4/Mult  precision=Full  arith_type="Signed  (2's comp)"  n_bits=18  bin_pt=17  quantization=Truncate  overflow=Wrap  en=off  latency=mult_latency  use_behavioral_HDL=on  opt=Speed  use_embedded=on  optimum_pipeline=off  pipeline=on  dbl_ovrd=off  use_rpm=off  placement_style=Rectangular shape  block_type=mult
  Mult1 : xbsIndex_r4/Mult  precision=Full  arith_type="Signed  (2's comp)"  n_bits=18  bin_pt=17  quantization=Truncate  overflow=Wrap  en=off  latency=mult_latency  use_behavioral_HDL=on  opt=Speed  use_embedded=on  optimum_pipeline=off  pipeline=on  dbl_ovrd=off  use_rpm=off  placement_style=Rectangular shape  block_type=mult
  Register{0..3} (4 alike) : xbsIndex_r4/Register  init=0  rst=off  en=on  dbl_ovrd=off  block_type=register
  coefficient : xbsIndex_r4/Constant  const=factor  gui_display_data_type=Fixed-point  arith_type=Signed (2's comp)  n_bits=coeff_bit_width  bin_pt=coeff_bin_pt  preci_type=Single  exp_width=8  frac_width=24  explicit_period=on  period=1  equ=P=C  opselect=C  inp2=PCIN>>17  opr=+  inp1=P  carry=CIN  dbl_ovrd=off  block_type=constant
  a_out : Outport
  b_out : Outport  Port=2
  c_out : Outport  Port=3
  d_out : Outport  Port=4
  real : Outport  Port=5
  imag : Outport  Port=6
  wires:
  Mult1/1 -> imag/1
  AddSub1/1 -> Mult1/2
  Mult0/1 -> real/1
  AddSub0/1 -> Mult0/2
  Register3/1 -> d_out/1
  coefficient/1 -> Mult1/1, Mult0/1
  Register2/1 -> c_out/1
  Register1/1 -> b_out/1
  Register0/1 -> a_out/1
  a/1 -> Register0/1, AddSub0/1
  b/1 -> Register1/1, AddSub1/1
  c/1 -> Register2/1, AddSub0/2
  d/1 -> Register3/1, AddSub1/2
  dv_in/1 -> Register3/2, Register2/2, Register1/2, Register0/2

== system s_c_nbe_m1k/DDC/dec_fir_async3/fir_col_async1/fir_tap2 ==
  a : Inport
  b : Inport  Port=2
  c : Inport  Port=3
  d : Inport  Port=4
  dv_in : Inport  Port=5
  AddSub0 : xbsIndex_r4/AddSub  mode=Addition  use_carryin=off  use_carryout=off  en=off  latency=add_latency  precision=Full  arith_type="Signed  (2's comp)"  n_bits=18  bin_pt=16  quantization=Truncate  overflow=Wrap  use_behavioral_HDL=on  hw_selection=Fabric  pipelined=off  use_rpm=on  dbl_ovrd=off  block_type=addsub
  AddSub1 : xbsIndex_r4/AddSub  mode=Addition  use_carryin=off  use_carryout=off  en=off  latency=add_latency  precision=Full  arith_type="Signed  (2's comp)"  n_bits=18  bin_pt=16  quantization=Truncate  overflow=Wrap  use_behavioral_HDL=on  hw_selection=Fabric  pipelined=off  use_rpm=on  dbl_ovrd=off  block_type=addsub
  Mult0 : xbsIndex_r4/Mult  precision=Full  arith_type="Signed  (2's comp)"  n_bits=18  bin_pt=17  quantization=Truncate  overflow=Wrap  en=off  latency=mult_latency  use_behavioral_HDL=on  opt=Speed  use_embedded=on  optimum_pipeline=off  pipeline=on  dbl_ovrd=off  use_rpm=off  placement_style=Rectangular shape  block_type=mult
  Mult1 : xbsIndex_r4/Mult  precision=Full  arith_type="Signed  (2's comp)"  n_bits=18  bin_pt=17  quantization=Truncate  overflow=Wrap  en=off  latency=mult_latency  use_behavioral_HDL=on  opt=Speed  use_embedded=on  optimum_pipeline=off  pipeline=on  dbl_ovrd=off  use_rpm=off  placement_style=Rectangular shape  block_type=mult
  Register{0..3} (4 alike) : xbsIndex_r4/Register  init=0  rst=off  en=on  dbl_ovrd=off  block_type=register
  coefficient : xbsIndex_r4/Constant  const=factor  gui_display_data_type=Fixed-point  arith_type=Signed (2's comp)  n_bits=coeff_bit_width  bin_pt=coeff_bin_pt  preci_type=Single  exp_width=8  frac_width=24  explicit_period=on  period=1  equ=P=C  opselect=C  inp2=PCIN>>17  opr=+  inp1=P  carry=CIN  dbl_ovrd=off  block_type=constant
  a_out : Outport
  b_out : Outport  Port=2
  c_out : Outport  Port=3
  d_out : Outport  Port=4
  real : Outport  Port=5
  imag : Outport  Port=6
  wires:
  Mult1/1 -> imag/1
  AddSub1/1 -> Mult1/2
  Mult0/1 -> real/1
  AddSub0/1 -> Mult0/2
  Register3/1 -> d_out/1
  coefficient/1 -> Mult1/1, Mult0/1
  Register2/1 -> c_out/1
  Register1/1 -> b_out/1
  Register0/1 -> a_out/1
  a/1 -> Register0/1, AddSub0/1
  b/1 -> Register1/1, AddSub1/1
  c/1 -> Register2/1, AddSub0/2
  d/1 -> Register3/1, AddSub1/2
  dv_in/1 -> Register0/2, Register1/2, Register3/2, Register2/2

== system s_c_nbe_m1k/DDC/dec_fir_async3/fir_col_async1/fir_tap3 ==
  a : Inport
  b : Inport  Port=2
  c : Inport  Port=3
  d : Inport  Port=4
  dv_in : Inport  Port=5
  AddSub0 : xbsIndex_r4/AddSub  mode=Addition  use_carryin=off  use_carryout=off  en=off  latency=add_latency  precision=Full  arith_type="Signed  (2's comp)"  n_bits=18  bin_pt=16  quantization=Truncate  overflow=Wrap  use_behavioral_HDL=on  hw_selection=Fabric  pipelined=off  use_rpm=on  dbl_ovrd=off  block_type=addsub
  AddSub1 : xbsIndex_r4/AddSub  mode=Addition  use_carryin=off  use_carryout=off  en=off  latency=add_latency  precision=Full  arith_type="Signed  (2's comp)"  n_bits=18  bin_pt=16  quantization=Truncate  overflow=Wrap  use_behavioral_HDL=on  hw_selection=Fabric  pipelined=off  use_rpm=on  dbl_ovrd=off  block_type=addsub
  Mult0 : xbsIndex_r4/Mult  precision=Full  arith_type="Signed  (2's comp)"  n_bits=18  bin_pt=17  quantization=Truncate  overflow=Wrap  en=off  latency=mult_latency  use_behavioral_HDL=on  opt=Speed  use_embedded=on  optimum_pipeline=off  pipeline=on  dbl_ovrd=off  use_rpm=off  placement_style=Rectangular shape  block_type=mult
  Mult1 : xbsIndex_r4/Mult  precision=Full  arith_type="Signed  (2's comp)"  n_bits=18  bin_pt=17  quantization=Truncate  overflow=Wrap  en=off  latency=mult_latency  use_behavioral_HDL=on  opt=Speed  use_embedded=on  optimum_pipeline=off  pipeline=on  dbl_ovrd=off  use_rpm=off  placement_style=Rectangular shape  block_type=mult
  Register{0..3} (4 alike) : xbsIndex_r4/Register  init=0  rst=off  en=on  dbl_ovrd=off  block_type=register
  coefficient : xbsIndex_r4/Constant  const=factor  gui_display_data_type=Fixed-point  arith_type=Signed (2's comp)  n_bits=coeff_bit_width  bin_pt=coeff_bin_pt  preci_type=Single  exp_width=8  frac_width=24  explicit_period=on  period=1  equ=P=C  opselect=C  inp2=PCIN>>17  opr=+  inp1=P  carry=CIN  dbl_ovrd=off  block_type=constant
  a_out : Outport
  b_out : Outport  Port=2
  c_out : Outport  Port=3
  d_out : Outport  Port=4
  real : Outport  Port=5
  imag : Outport  Port=6
  wires:
  Mult1/1 -> imag/1
  AddSub1/1 -> Mult1/2
  Mult0/1 -> real/1
  AddSub0/1 -> Mult0/2
  Register3/1 -> d_out/1
  coefficient/1 -> Mult1/1, Mult0/1
  Register2/1 -> c_out/1
  Register1/1 -> b_out/1
  Register0/1 -> a_out/1
  a/1 -> Register0/1, AddSub0/1
  b/1 -> Register1/1, AddSub1/1
  c/1 -> Register2/1, AddSub0/2
  d/1 -> Register3/1, AddSub1/2
  dv_in/1 -> Register0/2, Register1/2, Register3/2, Register2/2

== system s_c_nbe_m1k/DDC/dec_fir_async3/fir_col_async1/fir_tap4 ==
  a : Inport
  b : Inport  Port=2
  c : Inport  Port=3
  d : Inport  Port=4
  dv_in : Inport  Port=5
  AddSub0 : xbsIndex_r4/AddSub  mode=Addition  use_carryin=off  use_carryout=off  en=off  latency=add_latency  precision=Full  arith_type="Signed  (2's comp)"  n_bits=18  bin_pt=16  quantization=Truncate  overflow=Wrap  use_behavioral_HDL=on  hw_selection=Fabric  pipelined=off  use_rpm=on  dbl_ovrd=off  block_type=addsub
  AddSub1 : xbsIndex_r4/AddSub  mode=Addition  use_carryin=off  use_carryout=off  en=off  latency=add_latency  precision=Full  arith_type="Signed  (2's comp)"  n_bits=18  bin_pt=16  quantization=Truncate  overflow=Wrap  use_behavioral_HDL=on  hw_selection=Fabric  pipelined=off  use_rpm=on  dbl_ovrd=off  block_type=addsub
  Mult0 : xbsIndex_r4/Mult  precision=Full  arith_type="Signed  (2's comp)"  n_bits=18  bin_pt=17  quantization=Truncate  overflow=Wrap  en=off  latency=mult_latency  use_behavioral_HDL=on  opt=Speed  use_embedded=on  optimum_pipeline=off  pipeline=on  dbl_ovrd=off  use_rpm=off  placement_style=Rectangular shape  block_type=mult
  Mult1 : xbsIndex_r4/Mult  precision=Full  arith_type="Signed  (2's comp)"  n_bits=18  bin_pt=17  quantization=Truncate  overflow=Wrap  en=off  latency=mult_latency  use_behavioral_HDL=on  opt=Speed  use_embedded=on  optimum_pipeline=off  pipeline=on  dbl_ovrd=off  use_rpm=off  placement_style=Rectangular shape  block_type=mult
  Register{0..3} (4 alike) : xbsIndex_r4/Register  init=0  rst=off  en=on  dbl_ovrd=off  block_type=register
  coefficient : xbsIndex_r4/Constant  const=factor  gui_display_data_type=Fixed-point  arith_type=Signed (2's comp)  n_bits=coeff_bit_width  bin_pt=coeff_bin_pt  preci_type=Single  exp_width=8  frac_width=24  explicit_period=on  period=1  equ=P=C  opselect=C  inp2=PCIN>>17  opr=+  inp1=P  carry=CIN  dbl_ovrd=off  block_type=constant
  a_out : Outport
  b_out : Outport  Port=2
  c_out : Outport  Port=3
  d_out : Outport  Port=4
  real : Outport  Port=5
  imag : Outport  Port=6
  wires:
  Mult1/1 -> imag/1
  AddSub1/1 -> Mult1/2
  Mult0/1 -> real/1
  AddSub0/1 -> Mult0/2
  Register3/1 -> d_out/1
  coefficient/1 -> Mult1/1, Mult0/1
  Register2/1 -> c_out/1
  Register1/1 -> b_out/1
  Register0/1 -> a_out/1
  a/1 -> Register0/1, AddSub0/1
  b/1 -> Register1/1, AddSub1/1
  c/1 -> Register2/1, AddSub0/2
  d/1 -> Register3/1, AddSub1/2
  dv_in/1 -> Register3/2, Register2/2, Register1/2, Register0/2
